simulink model "fc3_abdin"  (R2026b)
settings: Solver=ode23t  StopTime=Tsim  MaxStep=4.0
PreLoadFcn:
  | fc3_abdin_parameters
values from neighbouring files (symbols this model uses):
  anode_tube_D = 0.01    [fc3_abdin_parameters.m]    (also in fc3_abdin_parameters2.m)
  env_p = 0.101325    [fc3_abdin_parameters.m]    (also in fc3_abdin_parameters2.m)
  I = linspace(0, 45.86, 100)    [fc3_abdin_parameters.m]    (also in fc3_abdin_parameters2.m = I_exp')
  N2_T = [-56.55, -50:10:-10, -5:1:5, 10:10:350]    [fc3_abdin_parameters.m]    (also in fc3_abdin_parameters2.m)
  p1 = 1.7320e-04    (= 0.0001732)    [fc3_abdin_parameters.m]    (also in fc3_abdin_parameters2.m)
  p2 = 1.0000e-11    (= 1e-11)    [fc3_abdin_parameters.m]    (also in fc3_abdin_parameters2.m)
  p3 = 0.0141    [fc3_abdin_parameters.m]    (also in fc3_abdin_parameters2.m)
  Stack_Pressure = 0.05    [fc3_abdin_parameters.m]    (also in fc3_abdin_parameters2.m)
  vector_time = linspace(0, Tsim, 100)    [fc3_abdin_parameters.m]    (also in fc3_abdin_parameters2.m = linspace(0, Tsim, length(I_exp)))
undefined symbols (not defined in the file or in its folder): FC_param
libraries: fl_lib x19, nesl_utility x6
settings Model: Creator=JakubEm  LastModifiedBy=JakubEm
settings DebuggingCC: AlgebraicLoopMsg=none
settings SimscapeCC: SimscapeLogType=all  SimscapeNominalValues="[{\"value\":\"1\",\"unit\":\"A\"},{\"value\":\"1\",\"unit\":\"bar\"},{\"value\":\"1\",\"unit\":\"cm^2\"},{\"value\":\"1\",\"unit\":\"cm^3/s\"},{\"value\":\"1\",\"unit\":\"kJ/kg\"},{\"value\":\"1\",\"unit\":\"kW\"},{\"value\":\"1\",\"unit\":\"l\"},{\"value\":\"1\",\"unit\":\"N\"},{\"value\":\"1\",\"unit\":\"N*m\"},{\"value\":\"1\",\"unit\":\"V\"},{\"value\":\"0.001\",\"unit\":\"Wb\"}]"  SimscapeUseEnergyAccounting=off

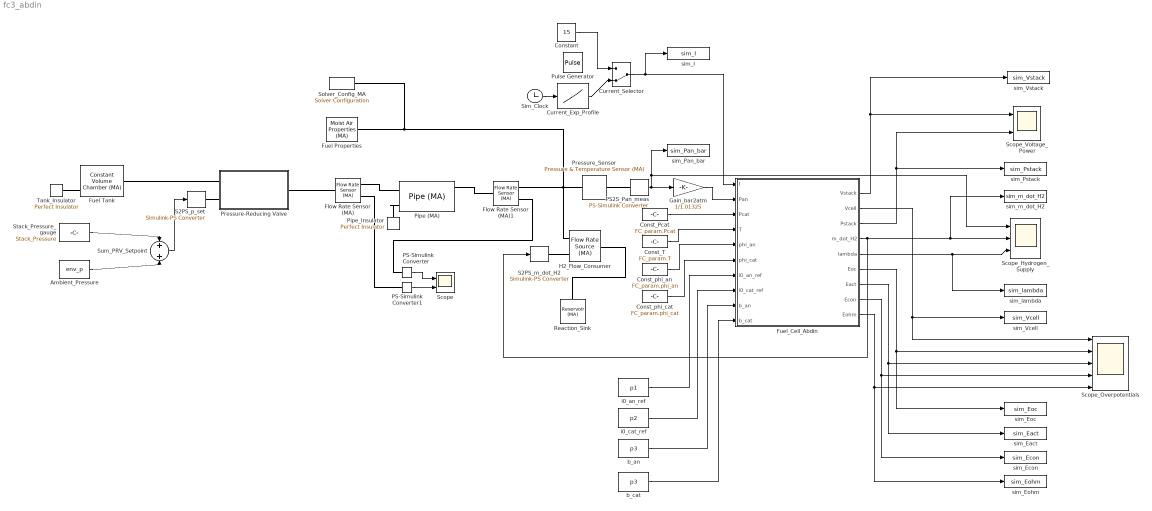
== system fc3_abdin ==
  Ambient_Pressure : Constant  Value=env_p
  Const_Pcat : Constant  Value=FC_param.Pcat
  Const_T : Constant  Value=FC_param.T
  Const_phi_an : Constant  Value=FC_param.phi_an
  Const_phi_cat : Constant  Value=FC_param.phi_cat
  Constant : Constant  Value=15
  Current_Exp_Profile : Lookup_n-D  NumberOfTableDimensions=1  BreakpointsForDimension1=vector_time  Table=I  InternalRulePriority=Speed  RndMeth=Simplest
  Current_Selector : ManualSwitch  CurrentSetting=0
  Flow Rate Sensor (MA) : fl_lib/Moist Air/Sensors/Flow Rate Sensor (MA)  mass_flow_measure=false  volumetric_flow_measure=true  volumetric_flow_conditions=foundation.enum.volumetric_flow_conditions.actual  p_std=0.101325 MPa  T_std=293.15 K  humidity_spec=foundation.enum.HumiditySpec.RelativeHumidity  RH_std=0.5  x_w_std=0.01  y_w_std=0.01  HR_std=0.01  Tw_std=287 K  trace_gas_spec=foundation.enum.trace_gas_spec.mass_fraction  x_g_std=0  y_g_std=0  RH_ws=1  energy_flow_measure=false  vapor_flow_measure=false  gas_flow_measure=false  droplets_flow_measure=false
  Flow Rate Sensor (MA)1 : fl_lib/Moist Air/Sensors/Flow Rate Sensor (MA)  mass_flow_measure=false  volumetric_flow_measure=true  volumetric_flow_conditions=foundation.enum.volumetric_flow_conditions.actual  p_std=0.101325 MPa  T_std=293.15 K  humidity_spec=foundation.enum.HumiditySpec.RelativeHumidity  RH_std=0.5  x_w_std=0.01  y_w_std=0.01  HR_std=0.01  Tw_std=287 K  trace_gas_spec=foundation.enum.trace_gas_spec.mass_fraction  x_g_std=0  y_g_std=0  RH_ws=1  energy_flow_measure=false  vapor_flow_measure=false  gas_flow_measure=false  droplets_flow_measure=false
  Fuel Properties : fl_lib/Moist Air/Utilities/Moist Air Properties (MA)  R_a=N2_R J/kg/K  T_TLU=N2_T degC  h_a_TLU=N2_h kJ/kg  mu_a_TLU=N2_mu s*uPa  k_a_TLU=N2_k mW/m/K  p_min=1 kPa  p_max=inf MPa  T_min=min(N2_T) degC  T_max=max(N2_T) degC  properties_range_check=simscape.enum.assert.action.error  p_atm=0.101325 MPa  T_atm=20 degC  enable_droplets=false  R_w=461.523 J/kg/K  p_ws_TLU=[1.71168953425982e-06; 3.93770601979424e-06; 1.28411717710344e-05; 3.80051394873809e-05; .00010323902900209; .000259873810798063; .000401741022116384; .000437454836117844; .000476040820618202; .000517704666185737; .000562664883741207; .000611212677444345; .000657088049117899; .000705987905898279; .000758082381149132; .000813549384183233; .000872574861129522; .00122818386934022; .0023392147667769; .00424668834054807; .00738442748706953; .0123512704340234; .0199458019246787; .0312006356960619; .0474147199263783; .0701823607447713; .10141797792131; .143375967241115; .198665399739302; .270259606559999; .361500961984849; .476101381081492; .618139196722055; .792053183687694; 1.0026345688121; 1.25501792086105; 1.55467186826983; 1.90739066433297; 2.31928772772542; 2.79679245576864; 3.34665187151016; 3.97593907083533; 4.69207105435535; 5.5028394740883; 6.41645928168037; 7.4416425436169; 8.58770832955728; 9.86474556030261; 11.2838558865497; 12.8575218898034; 14.6001810568052; 16.5291642526045] MPa  h_w_vap_TLU=[2836.88241275372; 2837.81392500514; 2838.63937175807; 2838.7309929628; 2838.06905313927; 2836.62597341095; 2835.60023952573; 2835.37006381376; 2835.13143158077; 2834.88429145066; 2834.62859062897; 2500.93420564316; 2498.55329907119; 2496.17495082036; 2493.79885912205; 2491.42474723191; 2489.05236104642; 2477.20875029194; 2453.54955988604; 2429.83856603313; 2406.00136954922; 2381.97406342174; 2357.69101156389; 2333.08088387814; 2308.06565480412; 2282.56034405021; 2256.47287422313; 2229.70428017508; 2202.14968030993; 2173.69998896199; 2144.24368406447; 2113.66758247452; 2081.85585110571; 2048.68725710494; 2014.03141249899; 1977.7449923284; 1939.66849592886; 1899.62342931686; 1857.40930169838; 1812.79975416601; 1765.53721731251; 1715.32525772152; 1661.81700477787; 1604.59703745016; 1543.1534616334; 1476.83692476464; 1404.80240352424; 1325.92091736114; 1238.61667822208; 1140.5102987018; 1027.62017777647; 892.733785613825] kJ/kg  h_w_TLU=[2396.55944251649; 2408.68643343608; 2427.1988031141; 2445.702165897; 2464.18429108356; 2482.62529466839; 2491.82135326629; 2493.6580151792; 2495.49372578218; 2497.32843835745; 2499.16210446923; 2500.99462758899; 2502.83092214066; 2504.6665223621; 2506.50140563013; 2508.335548891; 2510.16892865793; 2519.32352241995; 2537.56068088674; 2555.67742615292; 2573.6403223998; 2591.4109179101; 2608.9455037701; 2626.19492016262; 2643.10444358428; 2659.61377634497; 2675.58278696023; 2696.1846256545; 2716.49989553741; 2736.6235210957; 2756.61216047011; 2776.50561773853; 2796.33378922508; 2816.11979583049; 2835.88181423877; 2855.63430574511; 2875.38889327595; 2895.15500577172; 2914.94035964689; 2934.75132290228; 2954.59319330244; 2974.47041285505; 2994.38673458964; 3014.34535328009; 3034.34900867103; 3054.40006755764; 3074.50058946898; 3094.65237953784; 3114.85703128106; 3135.11596137801; 3155.43043805905; 3175.80160435813] kJ/kg  mu_w_TLU=[6.81365662228272; 7.04953750742707; 7.40970098298307; 7.76991278093907; 8.13017290129507; 8.49048134405107; 8.67065368632907; 8.70668960445667; 8.74272600580827; 8.77876289038387; 8.81480025818347; 8.85083810920707; 8.88687644345467; 8.92291526092627; 8.95895456162187; 8.99499434554147; 9.03103461268507; 9.21124319676307; 9.57169660671907; 9.93219833907507; 10.2927483938311; 10.6533467709871; 11.0139934705431; 11.3746884924991; 11.7354318368551; 12.0962235036111; 12.4570634927671; 12.8179518043231; 13.1788884382791; 13.5398733946351; 13.9009066733911; 14.2619882745471; 14.6231181981031; 14.9842964440591; 15.3455230124151; 15.7067979031711; 16.0681211163271; 16.4294926518831; 16.7909125098391; 17.1523806901951; 17.5138971929511; 17.8754620181071; 18.2370751656631; 18.5987366356191; 18.9604464279751; 19.3222045427311; 19.6840109798871; 20.0458657394431; 20.4077688213991; 20.7697202257551; 21.1317199525111; 21.4937680016671] s*uPa  k_w_TLU=[11.46288215976; 11.941997488935; 12.676358586935; 13.414208884935; 14.155548382935; 14.900377080935; 15.274099879935; 15.348949115735; 15.423833243535; 15.498752263335; 15.573706175135; 15.648694978935; 15.723718674735; 15.798777262535; 15.873870742335; 15.948999114135; 16.024162377935; 16.400502076935; 17.155798374935; 17.914583872935; 18.676858570935; 19.442622468935; 20.211875566935; 20.984617864935; 21.760849362935; 22.540570060935; 23.323779958935; 24.110479056935; 24.900667354935; 25.694344852935; 26.491511550935; 27.292167448935; 28.096312546935; 28.903946844935; 29.715070342935; 30.529683040935; 31.347784938935; 32.169376036935; 32.994456334935; 33.823025832935; 34.655084530935; 35.490632428935; 36.329669526935; 37.172195824935; 38.018211322935; 38.867716020935; 39.720709918935; 40.577193016935; 41.437165314935; 42.300626812935; 43.167577510935; 44.038017408935] mW/m/K  D_w=25 mm^2/s  trace_gas_model=foundation.enum.trace_gas_model.track_properties  R_g=H2_R J/kg/K  h_g_TLU=H2_h kJ/kg  mu_g_TLU=H2_mu s*uPa  k_g_TLU=H2_k mW/m/K  D_g=H2_D mm^2/s
      settings: AttributesFormatString=|
      | dry air --> N2
      | water vapor --> H2O
      | trace gas --> H2
  Fuel Tank : fl_lib/Moist Air/Elements/Constant Volume Chamber (MA)  volume=tank_V l  num_ports=foundation.enum.num_ports.one  area_A=pi*anode_tube_D^2/4 m^2  area_B=0.01 m^2  area_C=0.01 m^2  area_D=0.01 m^2  RH_ws=1  time_constant_cond=1e-3 s  time_constant_evap=1e-3 s  fraction_entrained=1  moisture_trace_gas_source=foundation.enum.moisture_trace_gas_source.none  moisture_source_spec=foundation.enum.MoistureSourceSpec.WaterVapor  vapor_from_liquid=false  moisture_mass_flow=0 kg/s  moisture_temperature_spec=foundation.enum.temperature_spec.atmospheric  moisture_temperature=293.15 K  trace_gas_mass_flow=0 kg/s  trace_gas_temperature_spec=foundation.enum.temperature_spec.atmospheric  trace_gas_temperature=293.15 K  p_init=tank_p bar  p_init_priority=foundation.enum.Priority.High  T_init=env_T degC  T_init_priority=foundation.enum.Priority.High  humidity_spec=foundation.enum.HumiditySpec.RelativeHumidity  RH_init=0  RH_init_priority=foundation.enum.Priority.High  x_w_init=0  x_w_init_priority=foundation.enum.Priority.None  y_w_init=0  y_w_init_priority=foundation.enum.Priority.None  HR_init=0  HR_init_priority=foundation.enum.Priority.None  Tw_init=287 K  Tw_init_priority=foundation.enum.Priority.High  trace_gas_spec=foundation.enum.trace_gas_spec.mole_fraction  x_g_init=0  x_g_init_priority=foundation.enum.Priority.None  y_g_init=tank_yH2  y_g_init_priority=foundation.enum.Priority.High  r_d_init=0  r_d_init_priority=foundation.enum.Priority.High
      settings: LogSimulationData=on
  Fuel_Cell_Abdin : Subsystem
  Gain_bar2atm : Gain  Gain=1/1.01325
  H2_Flow_Consumer : fl_lib/Moist Air/Sources/Flow Rate Source (MA)  source_type=foundation.enum.constant_controlled.controlled  flow_type=foundation.enum.mass_volumetric_flow.mass  mass_flow=0 kg/s  volumetric_flow=0 m^3/s  volumetric_flow_conditions=foundation.enum.volumetric_flow_conditions.standard  p_std=0.101325 MPa  T_std=293.15 K  humidity_spec=foundation.enum.HumiditySpec.RelativeHumidity  RH_std=0.5  x_w_std=0.01  y_w_std=0.01  HR_std=0.01  Tw_std=287 K  trace_gas_spec=foundation.enum.trace_gas_spec.mass_fraction  x_g_std=0  y_g_std=0  RH_ws=1  power_spec=foundation.enum.power_spec.isentropic  area_A=0.01 m^2  area_B=0.01 m^2
  PS-Simulink Converter : nesl_utility/PS-Simulink Converter  PhysicalDomain=network_engine_domain  SubClassName=ps_output  LeftPortType=input  RightPortType=output  PseudoPeriodic=off  Frequencies=[]  VectorFormat=inherit  Unit=inherit  AffineConversion=off
  PS-Simulink Converter1 : nesl_utility/PS-Simulink Converter  PhysicalDomain=network_engine_domain  SubClassName=ps_output  LeftPortType=input  RightPortType=output  PseudoPeriodic=off  Frequencies=[]  VectorFormat=inherit  Unit=inherit  AffineConversion=off
  PS2S_Pan_meas : nesl_utility/PS-Simulink Converter  PhysicalDomain=network_engine_domain  SubClassName=ps_output  LeftPortType=input  RightPortType=output  PseudoPeriodic=off  Frequencies=[]  VectorFormat=inherit  Unit=bar  AffineConversion=off
  Pipe (MA) : fl_lib/Moist Air/Elements/Pipe (MA)  length=1 m  area=pi*anode_tube_D^2/4 m^2  Dh=anode_tube_D m  length_add=0.1 m  roughness=15e-6 m  Re_lam=2000  Re_tur=4000  shape_factor=64  Nu_lam=3.66  wall_condensation=simscape.enum.onoff.off  RH_ws=1  time_constant_cond=1e-3 s  time_constant_evap=1e-3 s  fraction_entrained=1  moisture_trace_gas_source=foundation.enum.moisture_trace_gas_source.none  moisture_source_spec=foundation.enum.MoistureSourceSpec.WaterVapor  vapor_from_liquid=false  moisture_mass_flow=0 kg/s  moisture_temperature_spec=foundation.enum.temperature_spec.atmospheric  moisture_temperature=293.15 K  trace_gas_mass_flow=0 kg/s  trace_gas_temperature_spec=foundation.enum.temperature_spec.atmospheric  trace_gas_temperature=293.15 K  p_init=env_p MPa  p_init_priority=foundation.enum.Priority.High  T_init=env_T degC  T_init_priority=foundation.enum.Priority.High  humidity_spec=foundation.enum.HumiditySpec.RelativeHumidity  RH_init=0  RH_init_priority=foundation.enum.Priority.High  x_w_init=0  x_w_init_priority=foundation.enum.Priority.None  y_w_init=0  y_w_init_priority=foundation.enum.Priority.None  HR_init=0  HR_init_priority=foundation.enum.Priority.None  Tw_init=287 K  Tw_init_priority=foundation.enum.Priority.High  trace_gas_spec=foundation.enum.trace_gas_spec.mole_fraction  x_g_init=0  x_g_init_priority=foundation.enum.Priority.None  y_g_init=tank_yH2  y_g_init_priority=foundation.enum.Priority.High  r_d_init=0  r_d_init_priority=foundation.enum.Priority.High
      settings: LogSimulationData=on
  Pipe_Insulator : fl_lib/Thermal/Thermal Elements/Perfect Insulator  T_specify=off  T_priority=None  T=0 K  T_nominal_specify=off  T_nominal_value=1  T_nominal_unit=K
  Pressure-Reducing Valve : Subsystem  Tag=PublishSubsystem  mask(Pressure-Reducing Valve){D=anode_tube_D, r_min=1e-4, r_max=0.2, p_range=0.005}
      mask prompts: D "Connecting tube diameter (m)"; r_min "Min diameter ratio"; r_max "Max diameter ratio"; p_range "Pressure regulation range (MPa)"
      mask help: This subsystem models a pressure reducing valve that maintains a set pressure at port B. The valve is normally open. When the pressure is above the set pressure, it is fully closed.
  Pressure_Sensor : fl_lib/Moist Air/Sensors/Pressure & Temperature Sensor (MA)  reference=foundation.enum.MeasurementReference.absolute  pressure=true  pressure_spec=foundation.enum.PressureMeasementSpec.Absolute  temperature=false
      settings: LogSimulationData=on
  Pulse Generator : DiscretePulseGenerator  PulseType=Time based  Amplitude=15  Period=60  PulseWidth=5
  Reaction_Sink : fl_lib/Moist Air/Elements/Reservoir (MA)  reservoir_spec=foundation.enum.ReservoirSpec.StaticPressureTemperature  pressure_input=false  pressure_spec=foundation.enum.pressure_spec.atmospheric  reservoir_pressure=env_p MPa  temperature_input=false  temperature_spec=foundation.enum.temperature_spec.atmospheric  reservoir_temperature=env_T degC  humidity_input=false  humidity_spec=foundation.enum.HumiditySpec.RelativeHumidity  reservoir_RH=0.5  reservoir_x_w=0.01  reservoir_y_w=0.01  reservoir_HR=0.01  reservoir_Tw=287 K  trace_gas_input=false  trace_gas_spec=foundation.enum.trace_gas_spec.mass_fraction  reservoir_x_g=0.001  reservoir_y_g=0.001  water_droplets_input=false  reservoir_r_d=0  RH_ws=1  area_A=0.01 m^2  input_error_spec=foundation.enum.input_range_error.warn
  S2PS_m_dot_H2 : nesl_utility/Simulink-PS Converter  PhysicalDomain=network_engine_domain  SubClassName=ps_input  LeftPortType=input  RightPortType=output  PseudoPeriodic=off  Frequencies=[]  NoiseDistribution=none  NoiseParameters=[]  Unit=kg/s  AffineConversion=off  FilteringAndDerivatives=provide  SimscapeFilterOrder=1  InputFilterTimeConstant=0.001  UdotUserProvided=0
  S2PS_p_set : nesl_utility/Simulink-PS Converter  PhysicalDomain=network_engine_domain  SubClassName=ps_input  LeftPortType=input  RightPortType=output  PseudoPeriodic=off  Frequencies=[]  NoiseDistribution=none  NoiseParameters=[]  Unit=MPa  AffineConversion=off  FilteringAndDerivatives=provide  SimscapeFilterOrder=1  InputFilterTimeConstant=0.001  UdotUserProvided=0
  Scope : Scope  NumInputPorts=2
      settings: ActiveDisplayYMinimum=-0.004976538061549728  ActiveDisplayYMaximum=0.044788842553947557
  Scope_Hydrogen_Supply : Scope  NumInputPorts=3
      settings: ActiveDisplayYMinimum=-0.77250390624999965  ActiveDisplayYMaximum=6.9525351562499988
  Scope_Overpotentials : Scope  NumInputPorts=5
      settings: ActiveDisplayYMinimum=-0.15345493081287778  ActiveDisplayYMaximum=1.3810943773159003
  Scope_Voltage_Power : Scope  NumInputPorts=2
      settings: ActiveDisplayYMinimum=17.196754475233583  ActiveDisplayYMaximum=32.069622773534149
  Sim_Clock : Clock
  Solver_Config_MA : nesl_utility/Solver Configuration  PhysicalDomain=network_engine_domain  SubClassName=solver  LeftPortType=input  RightPortType=generic  Tones=[]  Harmonics=[]  SimulateNoise=off  Profile=off  UseLocalSampling=off  EnableSwitchedLinearOptims=on  FrequencyDomain=off  UseCCode=off  RelTol=0.001  AbsTol=1e-06  MinStep=1e-09  ToWorkspace=off  RevertToSquareIcSolve=off  NumHomotopyIterations=100  PhasorMode=off  PhasorModeNumHarmonics=1  ConsistencySolver=NEWTON_FTOL  CanonicalOrdering=UNORDERED  OptimizeIntermediates=UNOPTIMIZED  MulticoreSolverChoice=BACKWARD_EULER  IndexReductionMethod=DerivativeReplacement  DoDC=off  ResidualTolerance=1e-09  ConsistencyTolSource=GLOBAL  ConsistencyAbsTol=0.001  ConsistencyRelTol=0.001  ConsistencyTolFactor=0.001  UseLocalSolver=off  LocalSolverChoice=NE_BACKWARD_EULER_ADVANCER  ResolveIndetEquations=on  FunctionEvalNumThread=1  LocalSolverSampleTime=0.001  DoFixedCost=off  MaxNonlinIter=3  MaxModeIter=2  ComputeImpulses=off  ImpulseIterations=2  LinearAlgebra=auto  LinearAlgebraNumThread=0  EquationFormulation=NE_TIME_EF  DelaysMemoryBudget=1024  AutomaticFiltering=on  FilteringTimeConstant=0.001  PartitionStorageMethod=AS_NEEDED  PartitionMemoryBudget=1024  PartitionMethod=BALANCED  MultibodyUseLocalSolver=off  MultibodyLocalSolverChoice=ODE1  MultibodyLocalSolverSampleTime=0.001
  Stack_Pressure_gauge : Constant  Value=Stack_Pressure
  Sum_PRV_Setpoint : Sum
  Tank_Insulator : fl_lib/Thermal/Thermal Elements/Perfect Insulator  T_specify=off  T_priority=None  T=0 K  T_nominal_specify=off  T_nominal_value=1  T_nominal_unit=K
  b_an : Constant  Value=p3
  b_cat : Constant  Value=p3
  i0_an_ref : Constant  Value=p1
  i0_cat_ref : Constant  Value=p2
  sim_Eact : ToWorkspace  VariableName=sim_Eact  SampleTime=-1
  sim_Econ : ToWorkspace  VariableName=sim_Econ  SampleTime=-1
  sim_Eoc : ToWorkspace  VariableName=sim_Eoc  SampleTime=-1
  sim_Eohm : ToWorkspace  VariableName=sim_Eohm  SampleTime=-1
  sim_I : ToWorkspace  VariableName=sim_I  SampleTime=-1
  sim_Pan_bar : ToWorkspace  VariableName=sim_Pan_bar  SampleTime=-1
  sim_Pstack : ToWorkspace  VariableName=sim_Pstack  SampleTime=-1
  sim_Vcell : ToWorkspace  VariableName=sim_Vcell  SampleTime=-1
  sim_Vstack : ToWorkspace  VariableName=sim_Vstack  SampleTime=-1
  sim_lambda : ToWorkspace  VariableName=sim_lambda  SampleTime=-1
  sim_m_dot_H2 : ToWorkspace  VariableName=sim_m_dot_H2  SampleTime=-1
  wires:
  Stack_Pressure_gauge/1 -> Sum_PRV_Setpoint/1
  Ambient_Pressure/1 -> Sum_PRV_Setpoint/2
  Sum_PRV_Setpoint/1 -> S2PS_p_set/1
  PS2S_Pan_meas/1 -> sim_Pan_bar/1, Scope_Hydrogen_Supply/1, Gain_bar2atm/1
  Sim_Clock/1 -> Current_Exp_Profile/1
  Current_Exp_Profile/1 -> Current_Selector/2
  Current_Selector/1 -> Fuel_Cell_Abdin/1(I), sim_I/1
  Gain_bar2atm/1 -> Fuel_Cell_Abdin/2(Pan)
  Const_Pcat/1 -> Fuel_Cell_Abdin/3(Pcat)
  Const_T/1 -> Fuel_Cell_Abdin/4(T)
  Const_phi_an/1 -> Fuel_Cell_Abdin/5(phi_an)
  Const_phi_cat/1 -> Fuel_Cell_Abdin/6(phi_cat)
  Fuel_Cell_Abdin/4(m_dot_H2) -> sim_m_dot_H2/1, Scope_Hydrogen_Supply/2, S2PS_m_dot_H2/1
  Fuel_Cell_Abdin/1(Vstack) -> Scope_Voltage_Power/1, sim_Vstack/1
  Fuel_Cell_Abdin/3(Pstack) -> Scope_Voltage_Power/2, sim_Pstack/1
  Fuel_Cell_Abdin/2(Vcell) -> sim_Vcell/1, Scope_Overpotentials/1
  Fuel_Cell_Abdin/6(Eoc) -> sim_Eoc/1, Scope_Overpotentials/2
  Fuel_Cell_Abdin/7(Eact) -> sim_Eact/1, Scope_Overpotentials/3
  Fuel_Cell_Abdin/8(Econ) -> sim_Econ/1, Scope_Overpotentials/4
  Fuel_Cell_Abdin/9(Eohm) -> sim_Eohm/1, Scope_Overpotentials/5
  Fuel_Cell_Abdin/5(lambda) -> Scope_Hydrogen_Supply/3, sim_lambda/1
  PS-Simulink Converter/1 -> Scope/1
  PS-Simulink Converter1/1 -> Scope/2
  i0_an_ref/1 -> Fuel_Cell_Abdin/7(i0_an_ref)
  i0_cat_ref/1 -> Fuel_Cell_Abdin/8(i0_cat_ref)
  b_an/1 -> Fuel_Cell_Abdin/9(b_an)
  b_cat/1 -> Fuel_Cell_Abdin/10(b_cat)
  Constant/1 -> Current_Selector/1
  connections:
  S2PS_p_set/RConn1 -- Pressure-Reducing Valve/LConn2
  Fuel Tank/LConn1 -- Pressure-Reducing Valve/LConn1
  Fuel Tank/RConn3 -- Tank_Insulator/LConn1
  Pressure-Reducing Valve/RConn1 -- Flow Rate Sensor (MA)/LConn1
  Pipe (MA)/LConn2 -- Pipe_Insulator/LConn1
  Fuel Properties/RConn1 -- Flow Rate Sensor (MA)1/RConn1 -- H2_Flow_Consumer/LConn1 -- Pressure_Sensor/LConn1 -- Solver_Config_MA/RConn1
  Pressure_Sensor/RConn1 -- PS2S_Pan_meas/LConn1
  S2PS_m_dot_H2/RConn1 -- H2_Flow_Consumer/LConn2
  H2_Flow_Consumer/RConn1 -- Reaction_Sink/LConn1
  Flow Rate Sensor (MA)/RConn1 -- Pipe (MA)/LConn1
  Flow Rate Sensor (MA)1/LConn1 -- Pipe (MA)/RConn1
  PS-Simulink Converter/LConn1 -- Flow Rate Sensor (MA)1/RConn2
  Flow Rate Sensor (MA)/RConn2 -- PS-Simulink Converter1/LConn1

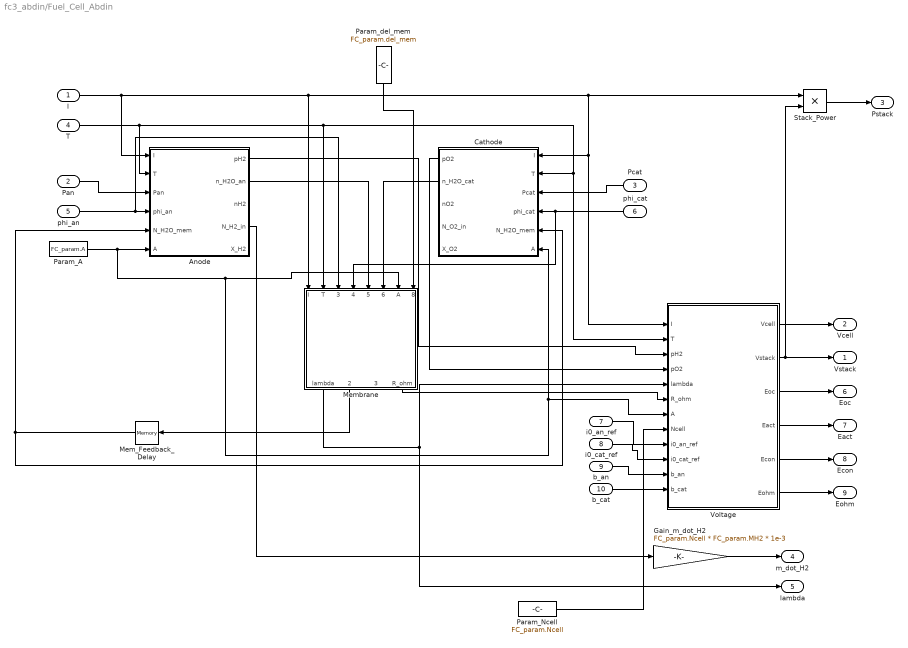
== system fc3_abdin/Fuel_Cell_Abdin ==
  I : Inport
  Pan : Inport  Port=2
  Pcat : Inport  Port=3
  T : Inport  Port=4
  phi_an : Inport  Port=5
  phi_cat : Inport  Port=6
  i0_an_ref : Inport  Port=7
  i0_cat_ref : Inport  Port=8
  b_an : Inport  Port=9
  b_cat : Inport  Port=10
  Anode : Subsystem
  Cathode : Subsystem
  Gain_m_dot_H2 : Gain  Gain=FC_param.Ncell * FC_param.MH2 * 1e-3
  Mem_Feedback_Delay : Memory
  Membrane : Subsystem
  Param_A : Constant  Value=FC_param.A
  Param_Ncell : Constant  Value=FC_param.Ncell
  Param_del_mem : Constant  Value=FC_param.del_mem
  Stack_Power : Product
  Voltage : Subsystem
  Vstack : Outport
  Vcell : Outport  Port=2
  Pstack : Outport  Port=3
  m_dot_H2 : Outport  Port=4
  lambda : Outport  Port=5
  Eoc : Outport  Port=6
  Eact : Outport  Port=7
  Econ : Outport  Port=8
  Eohm : Outport  Port=9
  wires:
  I/1 -> Cathode/1(I), Voltage/1(I), Stack_Power/1, Membrane/1(I), Anode/1(I)
  T/1 -> Voltage/2(T), Cathode/2(T), Membrane/2(T), Anode/2(T)
  Pan/1 -> Anode/3(Pan)
  phi_an/1 -> Anode/4(phi_an), Membrane/3(phi_an)
  Pcat/1 -> Cathode/3(Pcat)
  phi_cat/1 -> Membrane/4(phi_cat), Cathode/4(phi_cat)
  Param_A/1 -> Cathode/6(A), Voltage/7(A), Membrane/7(A), Anode/6(A)
  Param_del_mem/1 -> Membrane/8(del_mem)
  Param_Ncell/1 -> Voltage/8(Ncell)
  Anode/2(n_H2O_an) -> Membrane/5(n_H2O_an)
  Cathode/2(n_H2O_cat) -> Membrane/6(n_H2O_cat)
  Membrane/2(N_H2O_mem) -> Mem_Feedback_Delay/1
  Mem_Feedback_Delay/1 -> Anode/5(N_H2O_mem), Cathode/5(N_H2O_mem)
  Anode/1(pH2) -> Voltage/3(pH2)
  Cathode/1(pO2) -> Voltage/4(pO2)
  Membrane/1(lambda) -> Voltage/5(lambda), lambda/1
  Membrane/4(R_ohm) -> Voltage/6(R_ohm)
  Voltage/2(Vstack) -> Vstack/1, Stack_Power/2
  Anode/4(N_H2_in) -> Gain_m_dot_H2/1
  Voltage/1(Vcell) -> Vcell/1
  Stack_Power/1 -> Pstack/1
  Gain_m_dot_H2/1 -> m_dot_H2/1
  Voltage/3(Eoc) -> Eoc/1
  Voltage/4(Eact) -> Eact/1
  Voltage/5(Econ) -> Econ/1
  Voltage/6(Eohm) -> Eohm/1
  i0_an_ref/1 -> Voltage/9(i0_an_ref)
  i0_cat_ref/1 -> Voltage/10(i0_cat_ref)
  b_an/1 -> Voltage/11(b_an)
  b_cat/1 -> Voltage/12(b_cat)

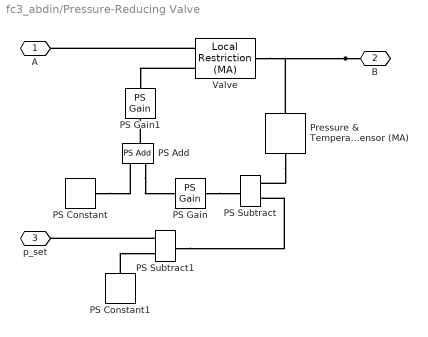
== system fc3_abdin/Pressure-Reducing Valve ==
  PS Add : fl_lib/Physical Signals/Functions/PS Add
  PS Constant : fl_lib/Physical Signals/Sources/PS Constant  constant=r_max^2
  PS Constant1 : fl_lib/Physical Signals/Sources/PS Constant  constant=p_range MPa
  PS Gain : fl_lib/Physical Signals/Functions/PS Gain  gain=(r_min^2 - r_max^2)/p_range 1/MPa
  PS Gain1 : fl_lib/Physical Signals/Functions/PS Gain  gain=pi*D^2/4 m^2
  PS Subtract : fl_lib/Physical Signals/Functions/PS Subtract
  PS Subtract1 : fl_lib/Physical Signals/Functions/PS Subtract
  Pressure & Temperature Sensor (MA) : fl_lib/Moist Air/Sensors/Pressure & Temperature Sensor (MA)  reference=foundation.enum.MeasurementReference.absolute  pressure=true  pressure_spec=foundation.enum.PressureMeasementSpec.Absolute  temperature=false
      settings: LogSimulationData=on
  Valve : fl_lib/Moist Air/Elements/Local Restriction (MA)  restriction_type=foundation.enum.restriction_type.variable  restriction_area=0.001 m^2  min_area=pi*(r_min*D)^2/4 m^2  max_area=pi*(r_max*D)^2/4 m^2  area=pi*D^2/4 m^2  Cd=0.64  B_lam=0.999
      settings: LogSimulationData=on
  A : PMIOPort  Side=Left
  B : PMIOPort  Port=2  Side=Right
  p_set : PMIOPort  Port=3  Side=Left
  connections:
  Valve/LConn2 -- PS Gain1/RConn1
  Pressure & Temperature Sensor (MA)/RConn1 -- PS Subtract/LConn1
  B/RConn1 -- Pressure & Temperature Sensor (MA)/LConn1 -- Valve/RConn1
  Valve/LConn1 -- A/RConn1
  PS Gain/LConn1 -- PS Subtract/RConn1
  PS Add/RConn1 -- PS Gain1/LConn1
  PS Add/LConn2 -- PS Gain/RConn1
  PS Constant/RConn1 -- PS Add/LConn1
  PS Subtract1/RConn1 -- PS Subtract/LConn2
  PS Subtract1/LConn1 -- p_set/RConn1
  PS Constant1/RConn1 -- PS Subtract1/LConn2

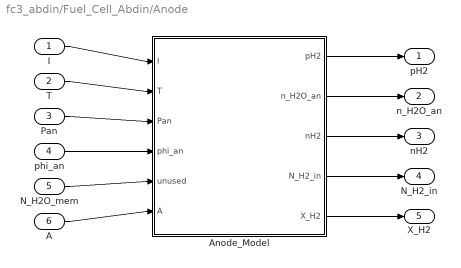
== system fc3_abdin/Fuel_Cell_Abdin/Anode ==
  I : Inport
  T : Inport  Port=2
  Pan : Inport  Port=3
  phi_an : Inport  Port=4
  N_H2O_mem : Inport  Port=5
  A : Inport  Port=6
  Anode_Model : MATLAB Function  TreatAsAtomicUnit=on
  pH2 : Outport
  n_H2O_an : Outport  Port=2
  nH2 : Outport  Port=3
  N_H2_in : Outport  Port=4
  X_H2 : Outport  Port=5
  wires:
  Anode_Model/4(N_H2_in) -> N_H2_in/1
  Anode_Model/3(nH2) -> nH2/1
  Anode_Model/2(n_H2O_an) -> n_H2O_an/1
  Anode_Model/1(pH2) -> pH2/1
  A/1 -> Anode_Model/6(A)
  N_H2O_mem/1 -> Anode_Model/5(unused)
  phi_an/1 -> Anode_Model/4(phi_an)
  Pan/1 -> Anode_Model/3(Pan)
  T/1 -> Anode_Model/2(T)
  I/1 -> Anode_Model/1(I)
  Anode_Model/5(X_H2) -> X_H2/1

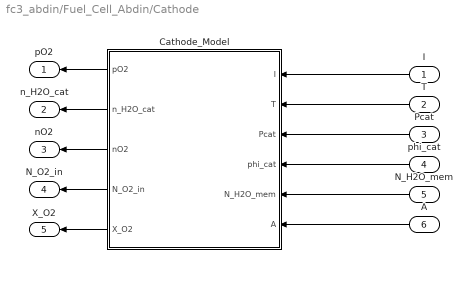
== system fc3_abdin/Fuel_Cell_Abdin/Cathode ==
  I : Inport
  T : Inport  Port=2
  Pcat : Inport  Port=3
  phi_cat : Inport  Port=4
  N_H2O_mem : Inport  Port=5
  A : Inport  Port=6
  Cathode_Model : MATLAB Function  TreatAsAtomicUnit=on
  pO2 : Outport
  n_H2O_cat : Outport  Port=2
  nO2 : Outport  Port=3
  N_O2_in : Outport  Port=4
  X_O2 : Outport  Port=5
  wires:
  Cathode_Model/4(N_O2_in) -> N_O2_in/1
  Cathode_Model/3(nO2) -> nO2/1
  Cathode_Model/2(n_H2O_cat) -> n_H2O_cat/1
  Cathode_Model/1(pO2) -> pO2/1
  A/1 -> Cathode_Model/6(A)
  N_H2O_mem/1 -> Cathode_Model/5(N_H2O_mem)
  phi_cat/1 -> Cathode_Model/4(phi_cat)
  Pcat/1 -> Cathode_Model/3(Pcat)
  T/1 -> Cathode_Model/2(T)
  I/1 -> Cathode_Model/1(I)
  Cathode_Model/5(X_O2) -> X_O2/1

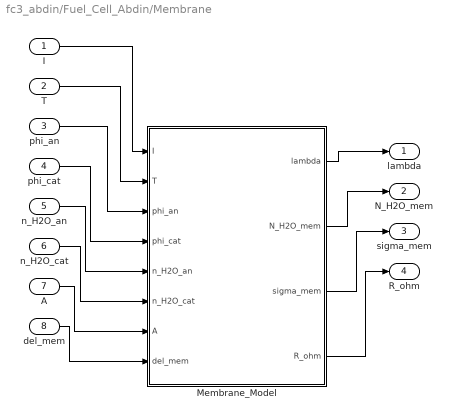
== system fc3_abdin/Fuel_Cell_Abdin/Membrane ==
  I : Inport
  T : Inport  Port=2
  phi_an : Inport  Port=3
  phi_cat : Inport  Port=4
  n_H2O_an : Inport  Port=5
  n_H2O_cat : Inport  Port=6
  A : Inport  Port=7
  del_mem : Inport  Port=8
  Membrane_Model : MATLAB Function  TreatAsAtomicUnit=on
  lambda : Outport
  N_H2O_mem : Outport  Port=2
  sigma_mem : Outport  Port=3
  R_ohm : Outport  Port=4
  wires:
  Membrane_Model/4(R_ohm) -> R_ohm/1
  Membrane_Model/3(sigma_mem) -> sigma_mem/1
  Membrane_Model/2(N_H2O_mem) -> N_H2O_mem/1
  Membrane_Model/1(lambda) -> lambda/1
  del_mem/1 -> Membrane_Model/8(del_mem)
  A/1 -> Membrane_Model/7(A)
  n_H2O_cat/1 -> Membrane_Model/6(n_H2O_cat)
  n_H2O_an/1 -> Membrane_Model/5(n_H2O_an)
  phi_cat/1 -> Membrane_Model/4(phi_cat)
  phi_an/1 -> Membrane_Model/3(phi_an)
  T/1 -> Membrane_Model/2(T)
  I/1 -> Membrane_Model/1(I)

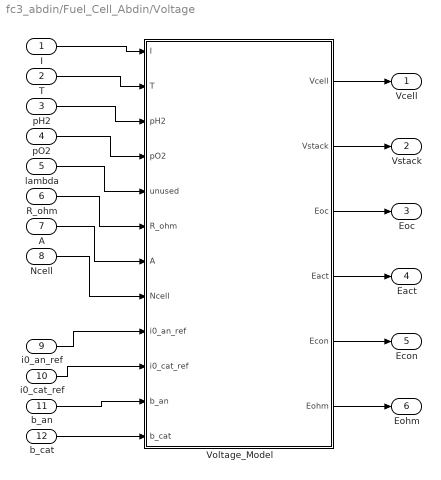
== system fc3_abdin/Fuel_Cell_Abdin/Voltage ==
  I : Inport
  T : Inport  Port=2
  pH2 : Inport  Port=3
  pO2 : Inport  Port=4
  lambda : Inport  Port=5
  R_ohm : Inport  Port=6
  A : Inport  Port=7
  Ncell : Inport  Port=8
  i0_an_ref : Inport  Port=9
  i0_cat_ref : Inport  Port=10
  b_an : Inport  Port=11
  b_cat : Inport  Port=12
  Voltage_Model : MATLAB Function  TreatAsAtomicUnit=on
  Vcell : Outport
  Vstack : Outport  Port=2
  Eoc : Outport  Port=3
  Eact : Outport  Port=4
  Econ : Outport  Port=5
  Eohm : Outport  Port=6
  wires:
  Voltage_Model/6(Eohm) -> Eohm/1
  Voltage_Model/5(Econ) -> Econ/1
  Voltage_Model/4(Eact) -> Eact/1
  Voltage_Model/3(Eoc) -> Eoc/1
  Voltage_Model/2(Vstack) -> Vstack/1
  Voltage_Model/1(Vcell) -> Vcell/1
  Ncell/1 -> Voltage_Model/8(Ncell)
  A/1 -> Voltage_Model/7(A)
  R_ohm/1 -> Voltage_Model/6(R_ohm)
  lambda/1 -> Voltage_Model/5(unused)
  pO2/1 -> Voltage_Model/4(pO2)
  pH2/1 -> Voltage_Model/3(pH2)
  T/1 -> Voltage_Model/2(T)
  I/1 -> Voltage_Model/1(I)
  i0_cat_ref/1 -> Voltage_Model/10(i0_cat_ref)
  i0_an_ref/1 -> Voltage_Model/9(i0_an_ref)
  b_an/1 -> Voltage_Model/11(b_an)
  b_cat/1 -> Voltage_Model/12(b_cat)

== matlab function fc3_abdin/Fuel_Cell_Abdin/Membrane/Membrane_Model ==
  data: I input; lambda output; T input; phi_an input; phi_cat input; n_H2O_an input; n_H2O_cat input; A input; del_mem input; N_H2O_mem output; sigma_mem output; R_ohm output
function [lambda, N_H2O_mem, sigma_mem, R_ohm] = Membrane_Model(I, T, phi_an, phi_cat, n_H2O_an, n_H2O_cat, A, del_mem)
%lambda = 0.0; N_H2O_mem = 0.0; sigma_mem = 0.0; R_ohm = 0.0;
% Membrane Ancillary (Abdin et al. 2016, Eqs. 28-49)
R = 8.3144; F = 96485; del_el = 0.008;
Dw = 1.28e-6; rhoH2O = 1.0; MH2O = 18.015;
Deff_an = 0.0403; Deff_cat = 0.0115;
i=I/A;
phi_avg = (phi_an + phi_cat)/2;
lambda = 0.043 + 17.18*phi_avg - 39.85*phi_avg^2 + 36.0*phi_avg^3;
nd = 2.5 * lambda / 22.0;
N_H2O_eod = nd * i / F;
C_H2O_ch = rhoH2O / MH2O;
C_H2O_mem_an = C_H2O_ch - (del_el * n_H2O_an) / Deff_an;
C_H2O_mem_cat = C_H2O_ch + (del_el * n_H2O_cat) / Deff_cat;
% C_H2_mem = (Pan * X_H2 / (R * T)) + 1e6 * (del_el * nH2 / Deff_an);
% C_O2_mem = (Pcat * X_O2 / (R * T)) + 1e6 * (del_el * nO2 / Deff_cat);
N_H2O_bd = (A * Dw / del_mem) * (C_H2O_mem_cat - C_H2O_mem_an);
N_H2O_mem = N_H2O_eod - N_H2O_bd;
sigma_mem = (0.005139 * lambda - 0.00326) * exp(1268 * (1/303 - 1/T));
R_ohm = del_mem / max(1e-4, sigma_mem);
end

== matlab function fc3_abdin/Fuel_Cell_Abdin/Anode/Anode_Model ==
  data: I input; pH2 output; T input; Pan input; phi_an input; unused input; A input; n_H2O_an output; nH2 output; N_H2_in output; X_H2 output
function [pH2, n_H2O_an, nH2, N_H2_in, X_H2] = Anode_Model(I, T, Pan, phi_an, ~, A)
%pH2 = 0.0; n_H2O_an = 0.0; nH2 = 0.0; N_H2_in = 0.0;
% Anode Ancillary (Abdin et al. 2016, Eqs. 3-16)
F = 96485; SH2 = 1.05;
T_C = T - 273.15;
log10_psat = -2.18 + 2.95e-2*T_C - 9.18e-5*T_C^2 + 1.44e-7*T_C^3;
psat = 10^log10_psat;
N_H2_cons = I / (2 * F);
N_H2_in = SH2 * N_H2_cons;
X_H2O_in = (phi_an * psat) / Pan;
N_H2O_in = N_H2_in * X_H2O_in / max(1e-4, (1 - X_H2O_in));
nH2 = N_H2_in / A;
n_H2O_an = N_H2O_in / A;
X_H2 = nH2 / max(1e-6, (nH2 + n_H2O_an));
pH2 = X_H2 * Pan;
end

== matlab function fc3_abdin/Fuel_Cell_Abdin/Cathode/Cathode_Model ==
  data: I input; pO2 output; T input; Pcat input; phi_cat input; N_H2O_mem input; A input; n_H2O_cat output; nO2 output; N_O2_in output; X_O2 output
function [pO2, n_H2O_cat, nO2, N_O2_in, X_O2] = Cathode_Model(I, T, Pcat, phi_cat, N_H2O_mem, A)
%pO2 = 0.0; n_H2O_cat = 0.0; nO2 = 0.0; N_O2_in = 0.0;
% Cathode Ancillary (Abdin et al. 2016, Eqs. 17-27)
F = 96485; SO2 = 20;
T_C = T - 273.15;
log10_psat = -2.18 + 2.95e-2*T_C - 9.18e-5*T_C^2 + 1.44e-7*T_C^3;
psat = 10^log10_psat;
N_O2_cons = I / (4 * F);
N_O2_in = SO2 * N_O2_cons;
N_H2O_in = N_O2_in * (phi_cat * psat) / max(1e-4, Pcat - phi_cat * psat);
N_H2O_gn = I / (2 * F);
N_H2O_tot = N_H2O_gn + N_H2O_mem + N_H2O_in;
nO2 = N_O2_in / A;
n_H2O_cat = N_H2O_tot / A;
X_O2 = nO2 / max(1e-6, (nO2 + n_H2O_cat));
pO2 = X_O2 * Pcat;
end

== matlab function fc3_abdin/Fuel_Cell_Abdin/Voltage/Voltage_Model ==
  data: I input; Vcell output; T input; pH2 input; pO2 input; unused input; R_ohm input; A input; Ncell input; i0_an_ref input; i0_cat_ref input; b_an input; b_cat input; Vstack output; Eoc output; Eact output; Econ output; Eohm output
function [Vcell, Vstack, Eoc, Eact, Econ, Eohm] = Voltage_Model(I, T, pH2, pO2, ~, R_ohm, A, Ncell, i0_an_ref, i0_cat_ref, b_an, b_cat)
% Voltage Ancillary (Abdin et al. 2016, Eqs. 50-85)
R = 8.3144; F = 96485; Tref = 298.15; E0rev = 1.229; dEdT = -0.9e-3;
dG_an = 29e3; dG_cat = 66e3; gamma_M = 47.0;
i = I / A; % current density [A/cm^2]
% 1. Nernst Open-Circuit Potential
Erev = E0rev + dEdT * (T - Tref);
Eoc = min(0.96, Erev + (R * T / (2 * F)) * log(max(1e-4, (pH2 * sqrt(max(1e-4, pO2))))));
% 2. Activation Overpotential (Tafel)
i0_an = gamma_M * exp(-dG_an / R * (1/T - 1/Tref)) * i0_an_ref;
i0_cat = gamma_M * exp(-dG_cat / R * (1/T - 1/Tref)) * i0_cat_ref;
if i > 0
    Eact_an = b_an * log10(max(1.0, i / i0_an));
    Eact_cat = b_cat * log10(max(1.0, i / i0_cat));
    Eact = Eact_an + Eact_cat;
else
    Eact = 0.0;
end
% 3. Ohmic Overpotential
Eohm = R_ohm * i;
% 4. Concentration Overpotential
iL = 0.9; % limiting current density [A/cm^2]
if i < iL
    Econ = -(R * T / (2 * F)) * log(max(1e-3, 1 - i / iL));
else
    Econ = 1.0;
end
Vcell = max(0.0, Eoc - Eact - Econ - Eohm);
Vstack = Ncell * Vcell;
end
